simulink model "demo_continuous"  (R2026a)
settings: Solver=ode4  StopTime=1  FixedStep=0.1
settings Model: Creator=harry_31916  LastModifiedBy=harry_31916

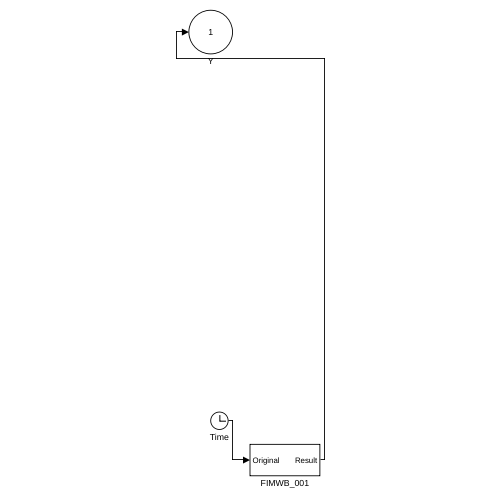
[thumbnail: Simulink's stored preview of the top-level diagram]
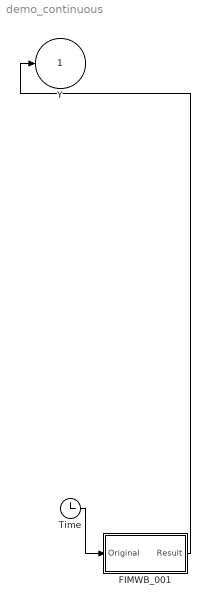
== system demo_continuous ==
  FIMWB_001 : Subsystem  Tag=fimwb.fault.1
  Time : Clock
  Y : Outport
  wires:
  Time/1 -> FIMWB_001/1(Original)
  FIMWB_001/1(Result) -> Y/1

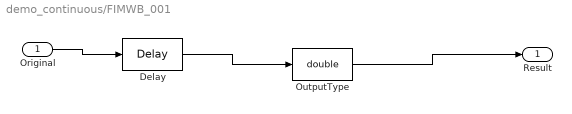
== system demo_continuous/FIMWB_001 ==
  Original : Inport
  Delay : TransportDelay  DelayTime=0.20000000000000001
  OutputType : DataTypeConversion  OutDataTypeStr=double  RndMeth=Round
  Result : Outport
  wires:
  Original/1 -> Delay/1
  Delay/1 -> OutputType/1
  OutputType/1 -> Result/1
